simulink model "emso_uotr_teste"  (Simulink 7.1)
settings: Solver=ode45  StartTime=0.0  StopTime=5  RelTol=1e-3
settings Model: Creator=lades  LastModifiedBy=W7
settings DataIOCC: ExternalInput=Az
settings DebuggingCC: SaveWithDisabledLinksMsg=none  SaveWithParameterizedLinksMsg=none  CheckSSInitialOutputMsg=off  SolverPrmCheckMsg=none  MultiTaskCondExecSysMsg=none  Int32ToFloatConvMsg=none  ModelReferenceDataLoggingMessage=none

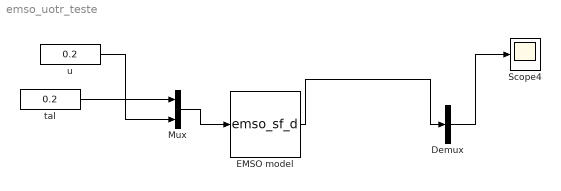
== system emso_uotr_teste ==
  Demux : Demux  Outputs=1
  EMSO model : S-Function  FunctionName=emso_sf_d  Parameters='emso_uotr.ems',2,1,0.5  EnableBusSupport=off
  Mux : Mux  Inputs=2
  Scope4 : Scope
      settings: TimeRange=5  YMin=0  YMax=45  SaveName=ScopeData3
  tal : Constant  Value=0.2  OutDataType=sfix(16)  OutScaling=2^0
  u : Constant  Value=0.2  OutDataType=sfix(16)  OutScaling=2^0
  wires:
  EMSO model/1 -> Demux/1
  Mux/1 -> EMSO model/1
  Demux/1 -> Scope4/1
  u/1 -> Mux/2
  tal/1 -> Mux/1
